simulink model "ex8pmdc"  (R2024b)
settings: Solver=VariableStepAuto  StartTime=0.0  StopTime=10.0  RelTol=1e-3
libraries: simulink x1
settings Model: Creator=pk309  LastModifiedBy=pk309

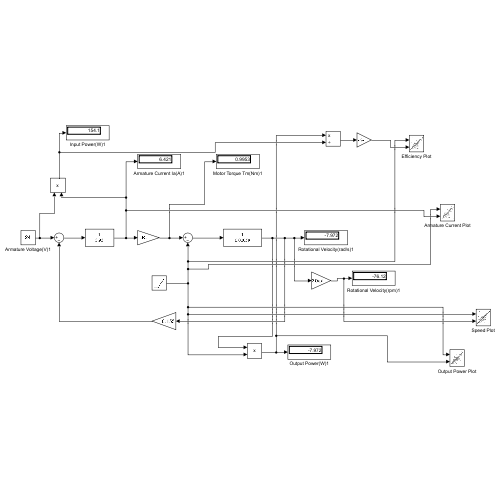
[thumbnail: Simulink's stored preview of the top-level diagram]
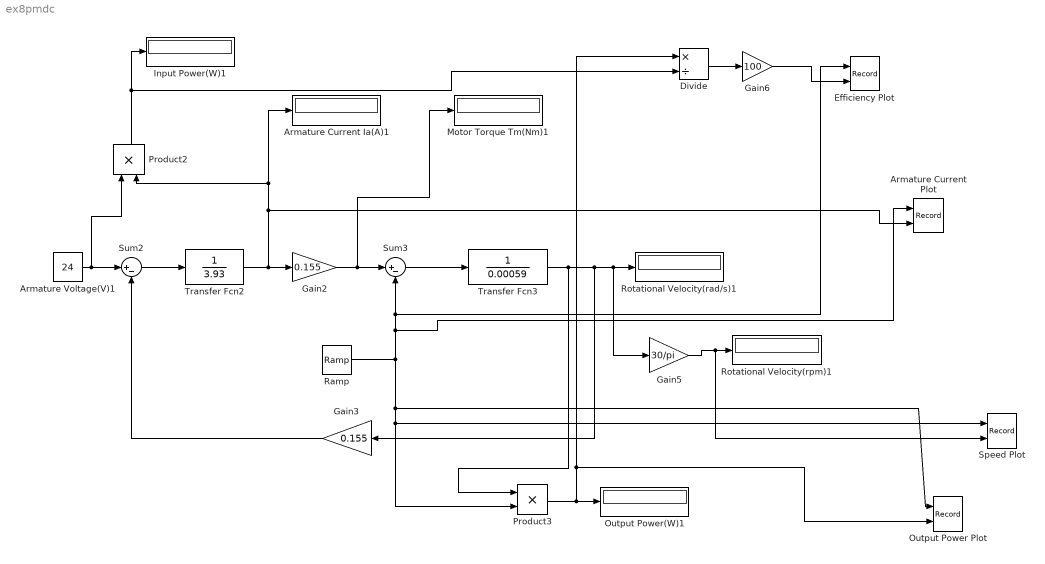
== system ex8pmdc ==
  Armature Current Ia(A)1 : Display
  "Armature Current Plot " : Record  FileSettingsInternal="{\"entries\":[{\"content\":{\"excelSettings\":{\"content\":{},\"type\":\"Streamout.ExcelSettings\"}},\"type\":\"Streamout.FileSettingStorage\",\"uuid\":\"\"}],\"packageUris\":[\"http:\\/\\/schema.mathworks.com\\/mf0\\/streamout_blocks\\/R2020a\"],\"version\":\"1.0\"}"  Layout=[1 1]  SignalsInternal="{\"entries\":[{\"content\":{},\"type\":\"RecordBlkView.InputSignals\",\"uuid\":\"\"}],\"packageUris\":[\"http:\\/\\/schema.mathworks.com\\/mf0\\/streamout_blocks\\/R2020a\"],\"version\":\"1.0\"}"  VisualizationBindings="{\"xyplotplugin\":{\"info\":[{\"series\":[{\"bindingParametersList\":[{\"parameter\":\"X-Axis\",\"signalID\":768,\"signalName\":\"Ramp\"},{\"parameter\":\"Y-Axis\",\"signalID\":772,\"signalName\":\"Transfer Fcn2\"}],\"seriesID\":0}],\"subplotID\":1}]}}"  CompatibilityTag=XY  st=-1
  Armature Voltage(V)1 : Constant  Value=24
  Divide : Product  Inputs=*/
  "Efficiency Plot " : Record  FileSettingsInternal="{\"entries\":[{\"content\":{\"excelSettings\":{\"content\":{},\"type\":\"Streamout.ExcelSettings\"}},\"type\":\"Streamout.FileSettingStorage\",\"uuid\":\"\"}],\"packageUris\":[\"http:\\/\\/schema.mathworks.com\\/mf0\\/streamout_blocks\\/R2020a\"],\"version\":\"1.0\"}"  Layout=[1 1]  SignalsInternal="{\"entries\":[{\"content\":{},\"type\":\"RecordBlkView.InputSignals\",\"uuid\":\"\"}],\"packageUris\":[\"http:\\/\\/schema.mathworks.com\\/mf0\\/streamout_blocks\\/R2020a\"],\"version\":\"1.0\"}"  VisualizationBindings="{\"xyplotplugin\":{\"info\":[{\"series\":[{\"bindingParametersList\":[{\"parameter\":\"X-Axis\",\"signalID\":776,\"signalName\":\"Ramp\"},{\"parameter\":\"Y-Axis\",\"signalID\":780,\"signalName\":\"Gain6\"}],\"seriesID\":0}],\"subplotID\":1}]}}"  CompatibilityTag=XY  st=-1
  Gain2 : Gain  Gain=0.155
  Gain3 : Gain  Gain=0.155
  Gain5 : Gain  Gain=30/pi
  Gain6 : Gain  Gain=100
  Input Power(W)1 : Display
  Motor Torque Tm(Nm)1 : Display
  Output Power Plot : Record  FileSettingsInternal="{\"entries\":[{\"content\":{\"excelSettings\":{\"content\":{},\"type\":\"Streamout.ExcelSettings\"}},\"type\":\"Streamout.FileSettingStorage\",\"uuid\":\"\"}],\"packageUris\":[\"http:\\/\\/schema.mathworks.com\\/mf0\\/streamout_blocks\\/R2020a\"],\"version\":\"1.0\"}"  Layout=[1 1]  SignalsInternal="{\"entries\":[{\"content\":{},\"type\":\"RecordBlkView.InputSignals\",\"uuid\":\"\"}],\"packageUris\":[\"http:\\/\\/schema.mathworks.com\\/mf0\\/streamout_blocks\\/R2020a\"],\"version\":\"1.0\"}"  VisualizationBindings="{\"xyplotplugin\":{\"info\":[{\"series\":[{\"bindingParametersList\":[{\"parameter\":\"X-Axis\",\"signalID\":784,\"signalName\":\"Ramp\"},{\"parameter\":\"Y-Axis\",\"signalID\":788,\"signalName\":\"Product3\"}],\"seriesID\":0}],\"subplotID\":1}]}}"  CompatibilityTag=XY  st=-1
  Output Power(W)1 : Display
  Product2 : Product
  Product3 : Product
  Ramp : simulink/Sources/Ramp  slope=0.1  start=0  InitialOutput=0
  Rotational Velocity(rad/s)1 : Display
  Rotational Velocity(rpm)1 : Display
  Speed Plot : Record  FileSettingsInternal="{\"entries\":[{\"content\":{\"excelSettings\":{\"content\":{},\"type\":\"Streamout.ExcelSettings\"}},\"type\":\"Streamout.FileSettingStorage\",\"uuid\":\"\"}],\"packageUris\":[\"http:\\/\\/schema.mathworks.com\\/mf0\\/streamout_blocks\\/R2020a\"],\"version\":\"1.0\"}"  Layout=[1 1]  SignalsInternal="{\"entries\":[{\"content\":{\"signals\":[{\"content\":{\"blockPath\":[],\"dimensions\":[1],\"domain\":\"\",\"lineColor\":\"#a2142f\",\"port\":1,\"sid\":[\"\"],\"signalID\":1,\"signalName\":\"Ramp\"},\"type\":\"RecordBlkView.Signal\",\"uuid\":\"\"},{\"content\":{\"blockPath\":[],\"dimensions\":[1],\"domain\":\"\",\"lineColor\":\"#139fff\",\"port\":2,\"sid\":[\"\"],\"signalID\":2,\"signalName\":\"Transfer Fcn2\"},\"type\":\"RecordBlkView.Signal\",\"uuid\":\"\"},{\"content\":{\"blockPath\":[],\"dimensions\":[1],\"domain\":\"\",\"lineColor\":\"#a2142f\",\"port\":1,\"sid\":[\"\"],\"signalID\":3,\"signalName\":\"Ramp\"},\"type\":\"RecordBlkView.Signal\",\"uuid\":\"\"},{\"content\":{\"blockPath\":[],\"dimensions\":[1],\"domain\":\"\",\"lineColor\":\"#139fff\",\"port\":2,\"sid\":[\"\"],\"signalID\":4,\"signalName\":\"Gain6\"},\"type\":\"RecordBlkView.Signal\",\"uuid\":\"\"},{\"content\":{\"blockPath\":[],\"dimensions\":[1],\"domain\":\"\",\"lineColor\":\"#a2142f\",\"port\":1,\"sid\":[\"\"],\"signalID\":5,\"signalName\":\"Ramp\"},\"type\":\"RecordBlkView.Signal\",\"uuid\":\"\"},{\"content\":{\"blockPath\":[],\"dimensions\":[1],\"domain\":\"\",\"lineColor\":\"#139fff\",\"port\":2,\"sid\":[\"\"],\"signalID\":6,\"signalName\":\"Product3\"},\"type\":\"RecordBlkView.Signal\",\"uuid\":\"\"},{\"content\":{\"blockPath\":[],\"dimensions\":[1],\"domain\":\"\",\"lineColor\":\"#a2142f\",\"plots\":[ 1 ],\"port\":1,\"sid\":[\"\"],\"signalID\":7,\"signalName\":\"Ramp\"},\"type\":\"RecordBlkView.Signal\",\"uuid\":\"\"},{\"content\":{\"blockPath\":[],\"dimensions\":[1],\"domain\":\"\",\"lineColor\":\"#139fff\",\"plots\":[ 1 ],\"port\":2,\"sid\":[\"\"],\"signalID\":8,\"signalName\":\"Gain5\"},\"type\":\"RecordBlkView.Signal\",\"uuid\":\"\"}]},\"type\":\"RecordBlkView.InputSignals\",\"uuid\":\"\"}],\"packageUris\":[\"http:\\/\\/schema.mathworks.com\\/mf0\\/streamout_blocks\\/R2020a\"],\"version\":\"1.0\"}"  VisualizationBindings="{\"xyplotplugin\":{\"info\":[{\"series\":[{\"bindingParametersList\":[{\"parameter\":\"X-Axis\",\"signalID\":7,\"signalName\":\"Ramp\"},{\"parameter\":\"Y-Axis\",\"signalID\":8,\"signalName\":\"Gain5\"}],\"seriesID\":0}],\"subplotID\":1}]}}"  CompatibilityTag=XY  st=-1
  Sum2 : Sum  Inputs=|+-
  Sum3 : Sum  Inputs=|+-
  Transfer Fcn2 : TransferFcn  Denominator=[0 3.93]
  Transfer Fcn3 : TransferFcn  Denominator=[0 0.00059]
  wires:
  Sum2/1 -> Transfer Fcn2/1
  Gain5/1 -> Speed Plot/2, Rotational Velocity(rpm)1/1
  Product2/1 -> Divide/2, Input Power(W)1/1
  Armature Voltage(V)1/1 -> Product2/1, Sum2/1
  Divide/1 -> Gain6/1
  Ramp/1 -> Output Power Plot/1, Speed Plot/1, Product3/2, "Efficiency Plot "/1, Sum3/2, "Armature Current Plot "/1
  Transfer Fcn2/1 -> Armature Current Ia(A)1/1, Product2/2, "Armature Current Plot "/2, Gain2/1
  Transfer Fcn3/1 -> Product3/1, Gain3/1, Gain5/1, Rotational Velocity(rad/s)1/1
  Sum3/1 -> Transfer Fcn3/1
  Gain6/1 -> "Efficiency Plot "/2
  Product3/1 -> Output Power Plot/2, Divide/1, Output Power(W)1/1
  Gain3/1 -> Sum2/2
  Gain2/1 -> Motor Torque Tm(Nm)1/1, Sum3/1
